simulink model "ex4"  (R2025b)
settings: Solver=VariableStepAuto  StartTime=0.0  StopTime=6  FixedStep=1e-4  RelTol=1e-5
values from neighbouring files (symbols this model uses):
  b_a = 2*K^2*(as*J-b)/(3*np^2*psi_nominal)    [sim4.m]
  I_base = sqrt(2) * K * I_n    [sim4.m]
  Id_ref = psi_nominal_pu*psi_base/L_M    [sim4.m]
  ki = ac*(R_s+R_R+R_a)    [sim4.m]
  kis = 2*K^2*as^2*J/(3*np^2*psi_nominal)    [sim4.m]
  kp = ac*L_sig    [sim4.m]
  kps = 2*K^2*as*J/(3*np^2*psi_nominal)    [sim4.m]
  L_M_est = L_M    (= 0.3354)    [sim4.m]
  L_sig = 0.0416    [sim4.m]
  R_a = ac*L_sig -(R_s+R_R)    [sim4.m]
  R_R = 2.106    [sim4.m]
  R_R_est = 2 * R_R    (= 4.212)    [sim4.m]
  V_base = sqrt(2) * K * V_n    [sim4.m]
  w_base = 2*pi*f_base    (= 314.159265359)    [sim4.m]
settings Model: Creator=Dimitris  LastModifiedBy=Dimitris
settings SolverCC: ZeroCrossAlgorithm=Adaptive
settings DebuggingCC: IgnoredZcDiagnostic=none

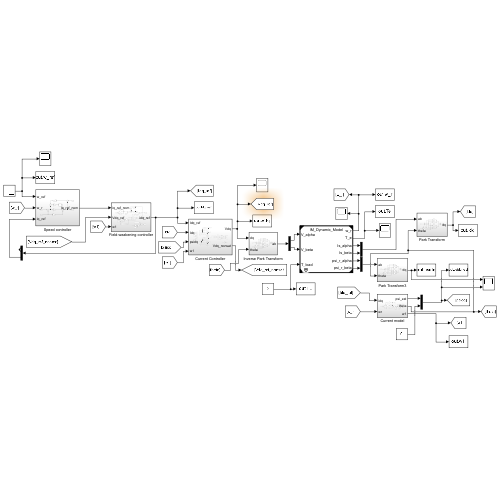
[thumbnail: Simulink's stored preview of the top-level diagram]
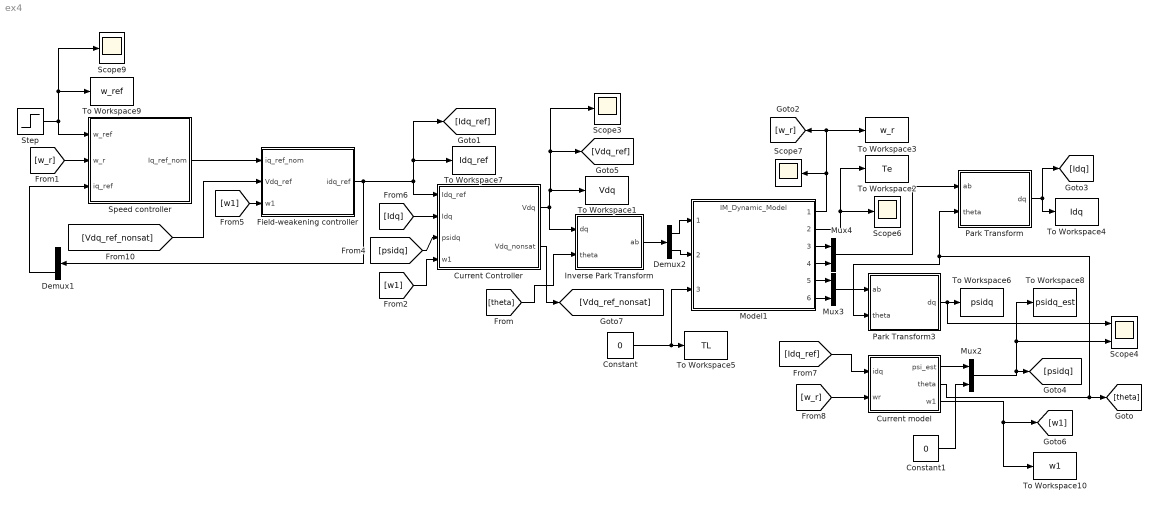
== system ex4 ==
  Constant : Constant  Value=0
  Constant1 : Constant  Value=0
  Current Controller : Subsystem
  Current model : Subsystem
  Demux1 : Demux  Outputs=2
  Demux2 : Demux  Outputs=2
  Field-weakening controller : Subsystem
  Inverse Park Transform : Subsystem
  Model1 : ModelReference  ModelNameDialog=IM_Dynamic_Model.slxp  ModelReferenceVersion=1.0  CopyOfModelProtected=on
  Mux2 : Mux  Inputs=2
  Mux3 : Mux  Inputs=2
  Mux4 : Mux  Inputs=2
  Park Transform : Subsystem
  Park Transform3 : Subsystem
  Scope{3,6..7,9} (4 alike) : Scope
      Scope3 settings: ActiveDisplayYMinimum=-383.16684608661609  ActiveDisplayYMaximum=403.91076310001017  DataLoggingVariableName=ScopeData3
      Scope6 settings: ActiveDisplayYMinimum=-5.6196905583497756  ActiveDisplayYMaximum=16.438809902973613
      Scope7 settings: ActiveDisplayYMinimum=-196.57703018378385  ActiveDisplayYMaximum=1769.193271654055  DataLoggingVariableName=ScopeData6
      Scope9 settings: ActiveDisplayYMinimum=137.44467859455347  ActiveDisplayYMaximum=333.79421944391549  DataLoggingVariableName=ScopeData8
  Scope4 : Scope  NumInputPorts=2
      settings: ActiveDisplayYMinimum=-0.12332605436153345  ActiveDisplayYMaximum=0.84755254408683534  DataLoggingVariableName=ScopeData4
  Speed controller : Subsystem
  Step : Step  Time=3.5  Before=5*w_base  After=3*w_base  SampleTime=0
  To Workspace1 : ToWorkspace  VariableName=Vdq  SaveFormat=Timeseries  SampleTime=-1
  To Workspace10 : ToWorkspace  VariableName=w1  SaveFormat=Timeseries  SampleTime=-1
  To Workspace2 : ToWorkspace  VariableName=Te  SaveFormat=Timeseries  SampleTime=-1
  To Workspace3 : ToWorkspace  VariableName=w_r  SaveFormat=Timeseries  SampleTime=-1
  To Workspace4 : ToWorkspace  VariableName=Idq  SaveFormat=Timeseries  SampleTime=-1
  To Workspace5 : ToWorkspace  VariableName=TL  SaveFormat=Timeseries  SampleTime=-1
  To Workspace6 : ToWorkspace  VariableName=psidq  SaveFormat=Timeseries  SampleTime=-1
  To Workspace7 : ToWorkspace  VariableName=Idq_ref  SaveFormat=Timeseries  SampleTime=-1
  To Workspace8 : ToWorkspace  VariableName=psidq_est  SaveFormat=Timeseries  SampleTime=-1
  To Workspace9 : ToWorkspace  VariableName=w_ref  SaveFormat=Timeseries  SampleTime=-1
  wires:
  Current Controller/1(Vdq) -> Inverse Park Transform/1(dq), Scope3/1, [Vdq_ref], To Workspace1/1
  Field-weakening controller/1(idq_ref) -> Current Controller/1(Idq_ref), To Workspace7/1, [Idq_ref], Demux1/1
  Inverse Park Transform/1(ab) -> Demux2/1
  Model1/4 -> Mux4/2
  Mux4/1 -> Park Transform/1(ab)
  Demux2/1 -> Model1/1
  Park Transform/1(dq) -> To Workspace4/1, [Idq]
  Mux3/1 -> Park Transform3/1(ab)
  Demux2/2 -> Model1/2
  Model1/3 -> Mux4/1
  Model1/2 -> To Workspace2/1, Scope6/1
  Model1/6 -> Mux3/2
  Park Transform3/1(dq) -> Scope4/1, To Workspace6/1
  Model1/1 -> [w_r], To Workspace3/1, Scope7/1
  Model1/5 -> Mux3/1
  [theta] -> Inverse Park Transform/2(theta)
  [psidq] -> Current Controller/3(psidq)
  [w1] -> Current Controller/4(w1)
  [w_r] -> Speed controller/2(w_r)
  Step/1 -> Speed controller/1(w_ref), To Workspace9/1, Scope9/1
  [Idq] -> Current Controller/2(Idq)
  [Idq_ref] -> Current model/1(idq)
  [w_r] -> Current model/2(wr)
  Mux2/1 -> [psidq], Scope4/2, To Workspace8/1
  [Vdq_ref_nonsat] -> Field-weakening controller/2(Vdq_ref)
  [w1] -> Field-weakening controller/3(w1)
  Demux1/2 -> Speed controller/3(iq_ref)
  Current Controller/2(Vdq_nonsat) -> [Vdq_ref_nonsat]
  Constant/1 -> Model1/3, To Workspace5/1
  Current model/1(psi_est) -> Mux2/1
  Current model/3(w1) -> To Workspace10/1, [w1]
  Current model/2(theta) -> Park Transform3/2(theta), Park Transform/2(theta), [theta]
  Constant1/1 -> Mux2/2
  Speed controller/1(Iq_ref_nom) -> Field-weakening controller/1(iq_ref_nom)

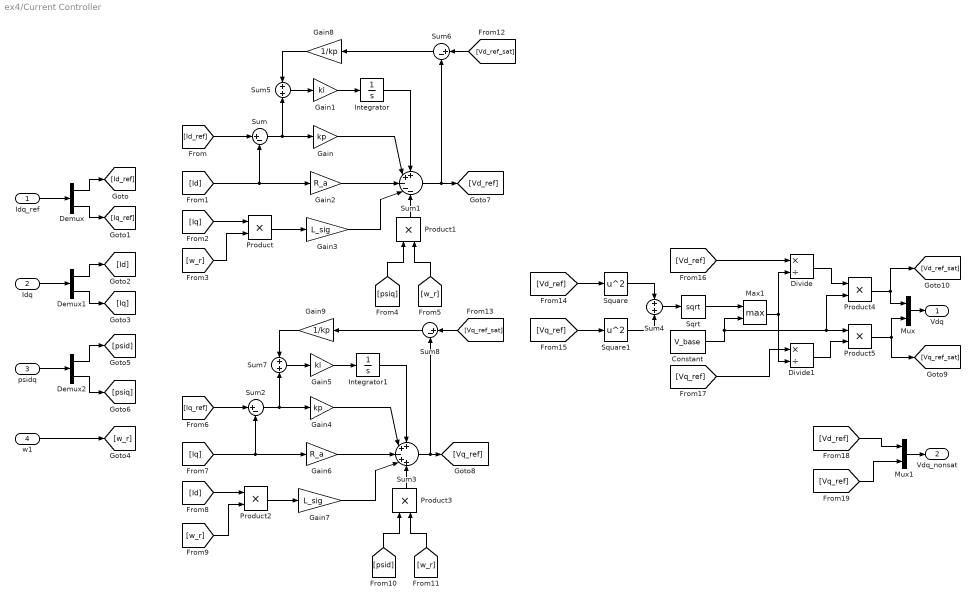
== system ex4/Current Controller ==
  Idq_ref : Inport
  Idq : Inport  Port=2
  psidq : Inport  Port=3
  w1 : Inport  Port=4
  Constant : Constant  Value=V_base
  Demux : Demux  Outputs=2
  Demux1 : Demux  Outputs=2
  Demux2 : Demux  Outputs=2
  Divide : Product  Inputs=*/
  Divide1 : Product  Inputs=*/
  Gain : Gain  Gain=kp
  Gain1 : Gain  Gain=ki
  Gain2 : Gain  Gain=R_a
  Gain3 : Gain  Gain=L_sig
  Gain4 : Gain  Gain=kp
  Gain5 : Gain  Gain=ki
  Gain6 : Gain  Gain=R_a
  Gain7 : Gain  Gain=L_sig
  Gain8 : Gain  Gain=1/kp
  Gain9 : Gain  Gain=1/kp
  Integrator : Integrator
  Integrator1 : Integrator
  Max1 : MinMax  Function=max  Inputs=2
  Mux : Mux  Inputs=2
  Mux1 : Mux  Inputs=2
  Product{,1..5} (6 alike) : Product
  Sqrt : Sqrt
  Square : Math  Operator=square
  Square1 : Math  Operator=square
  Sum{,2,6,8} (4 alike) : Sum  Inputs=|+-
  Sum1 : Sum  Inputs=++---
  Sum3 : Sum  Inputs=++-++
  Sum4 : Sum
  Sum5 : Sum
  Sum7 : Sum
  Vdq : Outport
  Vdq_nonsat : Outport  Port=2
  wires:
  Idq_ref/1 -> Demux/1
  Idq/1 -> Demux1/1
  Demux/1 -> [Id_ref]
  Demux/2 -> [Iq_ref]
  Demux1/1 -> [Id]
  Demux1/2 -> [Iq]
  [Id_ref] -> Sum/1
  [Id] -> Sum/2, Gain2/1
  Sum/1 -> Sum5/2, Gain/1
  Gain1/1 -> Integrator/1
  Integrator/1 -> Sum1/1
  Gain/1 -> Sum1/2
  Gain2/1 -> Sum1/3
  Gain3/1 -> Sum1/4
  Product/1 -> Gain3/1
  w1/1 -> [w_r]
  [Iq] -> Product/1
  [w_r] -> Product/2
  psidq/1 -> Demux2/1
  Demux2/1 -> [psid]
  Demux2/2 -> [psiq]
  [psiq] -> Product1/1
  [w_r] -> Product1/2
  Product1/1 -> Sum1/5
  Product3/1 -> Sum3/5
  [w_r] -> Product3/2
  [psid] -> Product3/1
  Product2/1 -> Gain7/1
  [Id] -> Product2/1
  Integrator1/1 -> Sum3/1
  Gain6/1 -> Sum3/3
  Gain5/1 -> Integrator1/1
  Gain7/1 -> Sum3/4
  Sum2/1 -> Sum7/2, Gain4/1
  [Iq_ref] -> Sum2/1
  [w_r] -> Product2/2
  [Iq] -> Sum2/2, Gain6/1
  Gain4/1 -> Sum3/2
  Sum1/1 -> [Vd_ref], Sum6/2
  [Vd_ref] -> Square/1
  [Vq_ref] -> Square1/1
  Square/1 -> Sum4/1
  Square1/1 -> Sum4/2
  Sum4/1 -> Sqrt/1
  Sqrt/1 -> Max1/1
  Max1/1 -> Divide/2, Divide1/2
  [Vd_ref] -> Divide/1
  [Vq_ref] -> Divide1/1
  Constant/1 -> Product4/2, Product5/1, Max1/2
  Mux/1 -> Vdq/1
  Sum5/1 -> Gain1/1
  Sum6/1 -> Gain8/1
  [Vd_ref_sat] -> Sum6/1
  Gain8/1 -> Sum5/1
  Sum7/1 -> Gain5/1
  Gain9/1 -> Sum7/1
  Sum3/1 -> Sum8/2, [Vq_ref]
  Sum8/1 -> Gain9/1
  [Vq_ref_sat] -> Sum8/1
  Divide/1 -> Product4/1
  Divide1/1 -> Product5/2
  Product5/1 -> [Vq_ref_sat], Mux/2
  Product4/1 -> [Vd_ref_sat], Mux/1
  Mux1/1 -> Vdq_nonsat/1
  [Vd_ref] -> Mux1/1
  [Vq_ref] -> Mux1/2

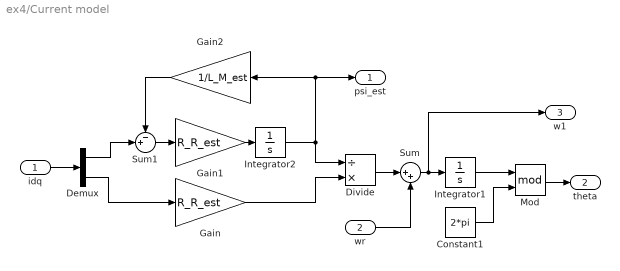
== system ex4/Current model ==
  idq : Inport
  wr : Inport  Port=2
  Constant1 : Constant  Value=2*pi
  Demux : Demux  Outputs=2
  Divide : Product  Inputs=/*
  Gain : Gain  Gain=R_R_est
  Gain1 : Gain  Gain=R_R_est
  Gain2 : Gain  Gain=1/L_M_est
  Integrator1 : Integrator
  Integrator2 : Integrator  InitialCondition=0.001
  Mod : Math  Operator=mod
  Sum : Sum  Inputs=|++
  Sum1 : Sum  Inputs=-+|
  psi_est : Outport
  theta : Outport  Port=2
  w1 : Outport  Port=3
  wires:
  Sum/1 -> w1/1, Integrator1/1
  Mod/1 -> theta/1
  Integrator1/1 -> Mod/1
  Constant1/1 -> Mod/2
  wr/1 -> Sum/2
  idq/1 -> Demux/1
  Demux/2 -> Gain/1
  Divide/1 -> Sum/1
  Gain/1 -> Divide/2
  Gain1/1 -> Integrator2/1
  Sum1/1 -> Gain1/1
  Demux/1 -> Sum1/2
  Gain2/1 -> Sum1/1
  Integrator2/1 -> Divide/1, psi_est/1, Gain2/1

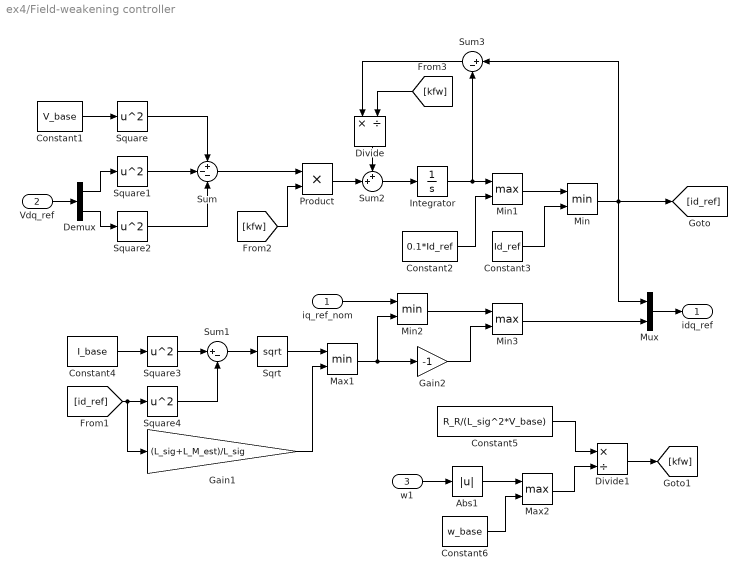
== system ex4/Field-weakening controller ==
  iq_ref_nom : Inport
  Vdq_ref : Inport  Port=2
  w1 : Inport  Port=3
  Abs1 : Abs  SaturateOnIntegerOverflow=off
  Constant1 : Constant  Value=V_base
  Constant2 : Constant  Value=0.1*Id_ref
  Constant3 : Constant  Value=Id_ref
  Constant4 : Constant  Value=I_base
  Constant5 : Constant  Value=R_R/(L_sig^2*V_base)
  Constant6 : Constant  Value=w_base
  Demux : Demux  Outputs=2
  Divide : Product  Inputs=*/
  Divide1 : Product  Inputs=*/
  Gain1 : Gain  Gain=(L_sig+L_M_est)/L_sig
  Gain2 : Gain  Gain=-1
  Integrator : Integrator
  Max1 : MinMax  Inputs=2
  Max2 : MinMax  Function=max  Inputs=2
  Min : MinMax  Inputs=2
  Min1 : MinMax  Function=max  Inputs=2
  Min2 : MinMax  Inputs=2
  Min3 : MinMax  Function=max  Inputs=2
  Mux : Mux  Inputs=2
  Product : Product
  Sqrt : Sqrt
  Square{,1..4} (5 alike) : Math  Operator=square
  Sum : Sum  Inputs=+--
  Sum1 : Sum  Inputs=|+-
  Sum2 : Sum  Inputs=++|
  Sum3 : Sum  Inputs=|+-
  idq_ref : Outport
  wires:
  Sum/1 -> Product/1
  Vdq_ref/1 -> Demux/1
  Constant1/1 -> Square/1
  Demux/1 -> Square1/1
  Demux/2 -> Square2/1
  Square/1 -> Sum/1
  Square1/1 -> Sum/2
  Square2/1 -> Sum/3
  Integrator/1 -> Sum3/2, Min1/1
  Constant2/1 -> Min1/2
  Constant3/1 -> Min/2
  Min1/1 -> Min/1
  iq_ref_nom/1 -> Min2/1
  Max1/1 -> Gain2/1, Min2/2
  Min/1 -> [id_ref], Sum3/1, Mux/1
  [id_ref] -> Square4/1, Gain1/1
  Sum1/1 -> Sqrt/1
  Constant4/1 -> Square3/1
  Square3/1 -> Sum1/1
  Square4/1 -> Sum1/2
  Min2/1 -> Min3/1
  Gain2/1 -> Min3/2
  Min3/1 -> Mux/2
  Mux/1 -> idq_ref/1
  Divide1/1 -> [kfw]
  Constant5/1 -> Divide1/1
  Constant6/1 -> Max2/2
  Max2/1 -> Divide1/2
  w1/1 -> Abs1/1
  Abs1/1 -> Max2/1
  [kfw] -> Product/2
  Sum2/1 -> Integrator/1
  Product/1 -> Sum2/2
  [kfw] -> Divide/2
  Sum3/1 -> Divide/1
  Divide/1 -> Sum2/1
  Sqrt/1 -> Max1/1
  Gain1/1 -> Max1/2

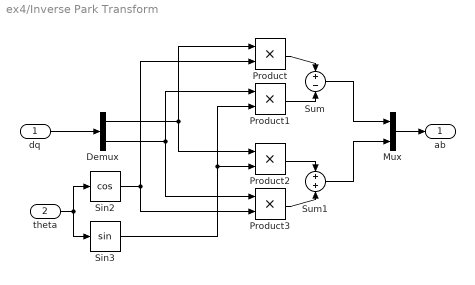
== system ex4/Inverse Park Transform ==
  dq : Inport
  theta : Inport  Port=2
  Demux : Demux  Outputs=2
  Mux : Mux  Inputs=2
  Product{,1..3} (4 alike) : Product
  Sin2 : Trigonometry  Operator=cos
  Sin3 : Trigonometry
  Sum : Sum  Inputs=+-
  Sum1 : Sum
  ab : Outport
  wires:
  Sum1/1 -> Mux/2
  Sin3/1 -> Product2/2, Product1/2
  Product1/1 -> Sum/2
  Demux/1 -> Product2/1, Product/1
  Mux/1 -> ab/1
  dq/1 -> Demux/1
  Sin2/1 -> Product/2, Product3/2
  Demux/2 -> Product1/1, Product3/1
  theta/1 -> Sin3/1, Sin2/1
  Sum/1 -> Mux/1
  Product/1 -> Sum/1
  Product3/1 -> Sum1/2
  Product2/1 -> Sum1/1

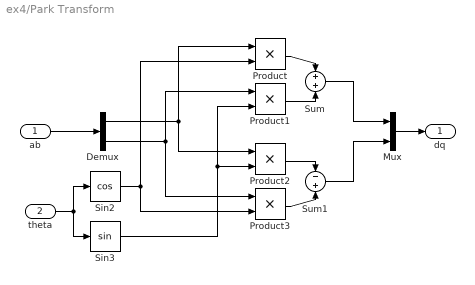
== system ex4/Park Transform ==
  ab : Inport
  theta : Inport  Port=2
  Demux : Demux  Outputs=2
  Mux : Mux  Inputs=2
  Product{,1..3} (4 alike) : Product
  Sin2 : Trigonometry  Operator=cos
  Sin3 : Trigonometry
  Sum : Sum
  Sum1 : Sum  Inputs=-+
  dq : Outport
  wires:
  Sin3/1 -> Product1/2, Product2/2
  Sin2/1 -> Product/2, Product3/2
  theta/1 -> Sin3/1, Sin2/1
  Demux/2 -> Product1/1, Product3/1
  Sum1/1 -> Mux/2
  Sum/1 -> Mux/1
  Demux/1 -> Product2/1, Product/1
  Product2/1 -> Sum1/1
  Product3/1 -> Sum1/2
  Product1/1 -> Sum/2
  Product/1 -> Sum/1
  Mux/1 -> dq/1
  ab/1 -> Demux/1

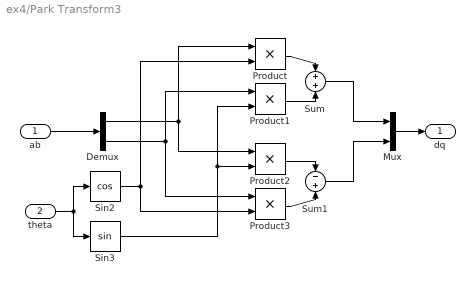
== system ex4/Park Transform3 ==
  ab : Inport
  theta : Inport  Port=2
  Demux : Demux  Outputs=2
  Mux : Mux  Inputs=2
  Product{,1..3} (4 alike) : Product
  Sin2 : Trigonometry  Operator=cos
  Sin3 : Trigonometry
  Sum : Sum
  Sum1 : Sum  Inputs=-+
  dq : Outport
  wires:
  Sin3/1 -> Product1/2, Product2/2
  Sin2/1 -> Product/2, Product3/2
  theta/1 -> Sin3/1, Sin2/1
  Demux/2 -> Product1/1, Product3/1
  Sum1/1 -> Mux/2
  Sum/1 -> Mux/1
  Demux/1 -> Product2/1, Product/1
  Product2/1 -> Sum1/1
  Product3/1 -> Sum1/2
  Product1/1 -> Sum/2
  Product/1 -> Sum/1
  Mux/1 -> dq/1
  ab/1 -> Demux/1

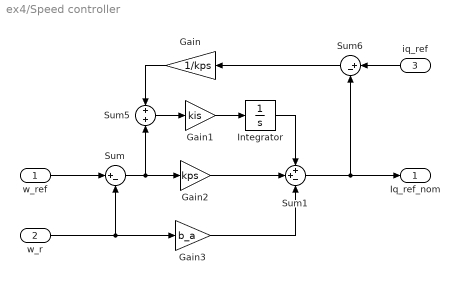
== system ex4/Speed controller ==
  w_ref : Inport
  w_r : Inport  Port=2
  iq_ref : Inport  Port=3
  Gain : Gain  Gain=1/kps
  Gain1 : Gain  Gain=kis
  Gain2 : Gain  Gain=kps
  Gain3 : Gain  Gain=b_a
  Integrator : Integrator
  Sum : Sum  Inputs=|+-
  Sum1 : Sum  Inputs=++-
  Sum5 : Sum
  Sum6 : Sum  Inputs=|+-
  Iq_ref_nom : Outport
  wires:
  Gain2/1 -> Sum1/2
  Gain/1 -> Sum5/1
  Sum5/1 -> Gain1/1
  Sum6/1 -> Gain/1
  w_ref/1 -> Sum/1
  w_r/1 -> Gain3/1, Sum/2
  Sum/1 -> Gain2/1, Sum5/2
  iq_ref/1 -> Sum6/1
  Sum1/1 -> Iq_ref_nom/1, Sum6/2
  Integrator/1 -> Sum1/1
  Gain3/1 -> Sum1/3
  Gain1/1 -> Integrator/1
